simulink model "grid_following_dqctrl"  (R2026b)
settings: Solver=VariableStepAuto
undefined symbols (not defined in the file or in its folder): param
libraries: nesl_utility x2, afe_ssc_lib x1
settings Model: Creator=d.bagnara  LastModifiedBy=d.bagnara

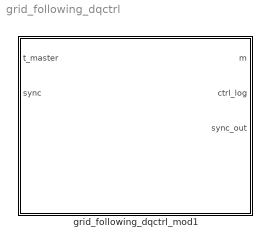
== system grid_following_dqctrl ==
  grid_following_dqctrl_mod1 : Subsystem  mask(Grid-following AFE (two-level bridge, LCL filter)){p=param.afe_follower(1)}
      mask prompts: p "Parameter struct p (afe_follower_module_param)"
      mask help: Grid-following AFE (DC-link voltage control, FHT-PLL) in one block: ideal two-level bridge, DC-link capacitor and LCL filter as a Simscape language component (afe_ssc.afe_two_level_lcl of afe_dq_single_block), control and PWM as one MATLAB Function (afe_follower_ctrl_pwm), measurements to the control through a Unit Delay of one tc (no algebraic loop). Interface of afe_dq_mod1 of grid_follower_dq.slx: ug_a/b/c left, Udc(+)/Udc(-) right, t_master in, M (14x1 pu) and ctrl_log (45x1) out. Master/slave: sync in and sync_out out, [i_xi_ref; i_eta_ref] in pu of ibez; with p.ctrl.slave = 1 the block runs its PLL and its current loops with the current references of the master (sync_out of the master to sync of the slave) and its DC-link loop is at rest, with p.ctrl.slave = 0 or absent it is a master and ignores sync. Parameter p: struct of private/afe_follower_module_param.m, e.g. param.afe_follower(1).
      mask Help: eval('pwrdoc = which(''grid_forming_following_afe.pdf''); if isempty(pwrdoc), pwrdoc = ''https://github.com/pwr-control/library/blob/main/library/documentation/grid_forming_following_afe/grid_forming_following_afe.pdf''; end; web(pwrdoc, ''-browser''); clear pwrdoc')
      mask Display:
      | port_label('LConn', 1, 'ug_a');
      | port_label('LConn', 2, 'ug_b');
      | port_label('LConn', 3, 'ug_c');
      | port_label('RConn', 1, 'Udc(+)');
      | port_label('RConn', 2, 'Udc(-)');
      | port_label('input', 1, 't_master');
      | port_label('input', 2, 'sync');
      | port_label('output', 1, 'M');
      | port_label('output', 2, 'ctrl_log');
      | port_label('output', 3, 'sync_out');

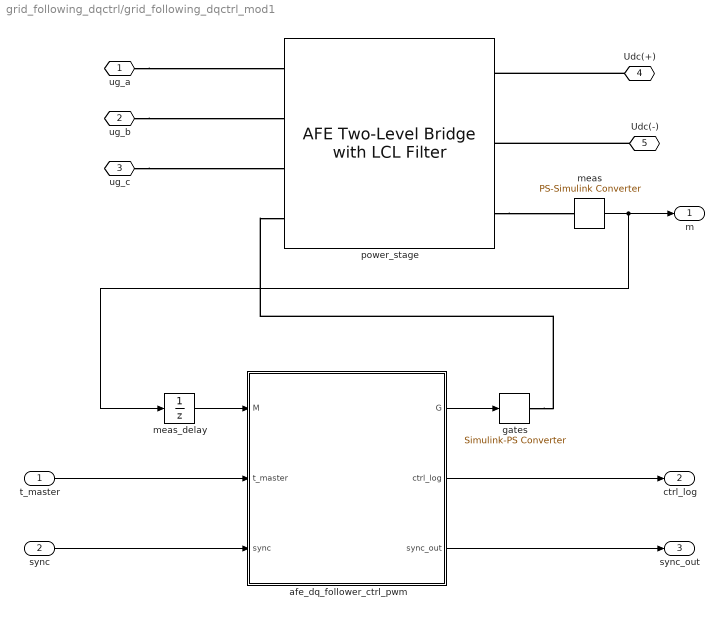
== system grid_following_dqctrl/grid_following_dqctrl_mod1 ==
  t_master : Inport
  sync : Inport  Port=2
  afe_dq_follower_ctrl_pwm : MATLAB Function  TreatAsAtomicUnit=on
  gates : nesl_utility/Simulink-PS Converter  PhysicalDomain=network_engine_domain  SubClassName=ps_input  LeftPortType=input  RightPortType=output  PseudoPeriodic=off  Frequencies=[]  NoiseDistribution=none  NoiseParameters=[]  Unit=V  AffineConversion=off  FilteringAndDerivatives=provide  SimscapeFilterOrder=1  InputFilterTimeConstant=0.001  UdotUserProvided=0
  meas : nesl_utility/PS-Simulink Converter  PhysicalDomain=network_engine_domain  SubClassName=ps_output  LeftPortType=input  RightPortType=output  PseudoPeriodic=off  Frequencies=[]  VectorFormat=inherit  Unit=1  AffineConversion=off
  meas_delay : UnitDelay  SampleTime=p.pwm.tc
  power_stage : afe_ssc_lib/AFE Two-Level Bridge with LCL Filter  Vth=p.hw.Vth V  Ron=p.hw.Ron Ohm  Goff=p.hw.Goff 1/Ohm  cap_dc=afe_ssc.onoff.on  Cdc=p.hw.Cdc F  Rdc=p.hw.Rdc Ohm  L1p=p.hw.L1p H  L10=p.hw.L10 H  R1=p.hw.R1 Ohm  Lls1=p.hw.Lls1 H  Cf=p.hw.Cf F  Rcf=p.hw.Rcf Ohm  L2p=p.hw.L2p H  L20=p.hw.L20 H  R2=p.hw.R2 Ohm  Lls2=p.hw.Lls2 H  ubez=p.hw.ubez V  ibez=p.hw.ibez A  udc_nom=p.hw.udc_nom V  vdc_specify=off  vdc_priority=None  vdc=0 V  vdc_nominal_specify=off  vdc_nominal_value=1  vdc_nominal_unit=V  vcap_specify=off  vcap_priority=None  vcap=0 V  vcap_nominal_specify=off  vcap_nominal_value=1  vcap_nominal_unit=V  ic_specify=off  ic_priority=None  ic=0 A  ic_nominal_specify=off  ic_nominal_value=1  ic_nominal_unit=A  vm_a_specify=off  vm_a_priority=None  vm_a=0 V  vm_a_nominal_specify=off  vm_a_nominal_value=1  vm_a_nominal_unit=V  vm_b_specify=off  vm_b_priority=None  vm_b=0 V  vm_b_nominal_specify=off  vm_b_nominal_value=1  vm_b_nominal_unit=V  vm_c_specify=off  vm_c_priority=None  vm_c=0 V  vm_c_nominal_specify=off  vm_c_nominal_value=1  vm_c_nominal_unit=V  i_ah_specify=off  i_ah_priority=None  i_ah=0 A  i_ah_nominal_specify=off  i_ah_nominal_value=1  i_ah_nominal_unit=A  i_al_specify=off  i_al_priority=None  i_al=0 A  i_al_nominal_specify=off  i_al_nominal_value=1  i_al_nominal_unit=A  i_bh_specify=off  i_bh_priority=None  i_bh=0 A  i_bh_nominal_specify=off  i_bh_nominal_value=1  i_bh_nominal_unit=A  i_bl_specify=off  i_bl_priority=None  i_bl=0 A  i_bl_nominal_specify=off  i_bl_nominal_value=1  i_bl_nominal_unit=A  i_ch_specify=off  i_ch_priority=None  i_ch=0 A  i_ch_nominal_specify=off  i_ch_nominal_value=1  i_ch_nominal_unit=A  i_cl_specify=off  i_cl_priority=None  i_cl=0 A  i_cl_nominal_specify=off  i_cl_nominal_value=1  i_cl_nominal_unit=A  i1_a_specify=off  i1_a_priority=None  i1_a=0 A  i1_a_nominal_specify=off  i1_a_nominal_value=1  i1_a_nominal_unit=A  i1_b_specify=off  i1_b_priority=None  i1_b=0 A  i1_b_nominal_specify=off  i1_b_nominal_value=1  i1_b_nominal_unit=A  i1_c_specify=off  i1_c_priority=None  i1_c=0 A  i1_c_nominal_specify=off  i1_c_nominal_value=1  i1_c_nominal_unit=A  vk_a_specify=off  vk_a_priority=None  vk_a=0 V  vk_a_nominal_specify=off  vk_a_nominal_value=1  vk_a_nominal_unit=V  vk_b_specify=off  vk_b_priority=None  vk_b=0 V  vk_b_nominal_specify=off  vk_b_nominal_value=1  vk_b_nominal_unit=V  vk_c_specify=off  vk_c_priority=None  vk_c=0 V  vk_c_nominal_specify=off  vk_c_nominal_value=1  vk_c_nominal_unit=V  vn_specify=off  vn_priority=None  vn=0 V  vn_nominal_specify=off  vn_nominal_value=1  vn_nominal_unit=V  vc_a_specify=off  vc_a_priority=None  vc_a=0 V  vc_a_nominal_specify=off  vc_a_nominal_value=1  vc_a_nominal_unit=V  vc_b_specify=off  vc_b_priority=None  vc_b=0 V  vc_b_nominal_specify=off  vc_b_nominal_value=1  vc_b_nominal_unit=V  vc_c_specify=off  vc_c_priority=None  vc_c=0 V  vc_c_nominal_specify=off  vc_c_nominal_value=1  vc_c_nominal_unit=V  i2_a_specify=off  i2_a_priority=None  i2_a=0 A  i2_a_nominal_specify=off  i2_a_nominal_value=1  i2_a_nominal_unit=A  i2_b_specify=off  i2_b_priority=None  i2_b=0 A  i2_b_nominal_specify=off  i2_b_nominal_value=1  i2_b_nominal_unit=A  i2_c_specify=off  i2_c_priority=None  i2_c=0 A  i2_c_nominal_specify=off  i2_c_nominal_value=1  i2_c_nominal_unit=A  j_ab_specify=off  j_ab_priority=None  j_ab=0 A  j_ab_nominal_specify=off  j_ab_nominal_value=1  j_ab_nominal_unit=A  j_bc_specify=off  j_bc_priority=None  j_bc=0 A  j_bc_nominal_specify=off  j_bc_nominal_value=1  j_bc_nominal_unit=A
  ug_a : PMIOPort  Side=Left
  ug_b : PMIOPort  Port=2  Side=Left
  ug_c : PMIOPort  Port=3  Side=Left
  Udc(+) : PMIOPort  Port=4  Side=Right
  Udc(-) : PMIOPort  Port=5  Side=Right
  m : Outport
  ctrl_log : Outport  Port=2
  sync_out : Outport  Port=3
  wires:
  t_master/1 -> afe_dq_follower_ctrl_pwm/2(t_master)
  meas/1 -> m/1, meas_delay/1
  meas_delay/1 -> afe_dq_follower_ctrl_pwm/1(M)
  afe_dq_follower_ctrl_pwm/1(G) -> gates/1
  afe_dq_follower_ctrl_pwm/2(ctrl_log) -> ctrl_log/1
  sync/1 -> afe_dq_follower_ctrl_pwm/3(sync)
  afe_dq_follower_ctrl_pwm/3(sync_out) -> sync_out/1
  connections:
  gates/RConn1 -- power_stage/LConn4
  power_stage/RConn3 -- meas/LConn1
  ug_a/RConn1 -- power_stage/LConn1
  ug_b/RConn1 -- power_stage/LConn2
  ug_c/RConn1 -- power_stage/LConn3
  Udc(+)/RConn1 -- power_stage/RConn1
  Udc(-)/RConn1 -- power_stage/RConn2

== matlab function grid_following_dqctrl/grid_following_dqctrl_mod1/afe_dq_follower_ctrl_pwm ==
  settings: updateMethod=DISCRETE  sampleTime=p.pwm.tc
  data: M input; G output; t_master input; sync input size=[2 1]; ctrl_log output; p parameter; sync_out output size=[2 1]
function [G, ctrl_log, sync_out] = afe_follower_ctrl_pwm(M, t_master, sync, p)
%AFE_FOLLOWER_CTRL_PWM  Control and PWM of one grid-following AFE (DC-link voltage control) in one MATLAB Function block.
%#codegen
%
%   [G, ctrl_log, sync_out] = afe_follower_ctrl_pwm(M, t_master, sync, p)
%
%   Equivalent of afe_dq_mod1/AFE_control (triggered subsystem afe_control) plus afe/sv_pwm (carrier,
%   TRGO, gate commands) of grid_follower_dq.slx (R2026b, commit 3fa4567), written as one function so
%   that the control of one AFE counts as ONE nonvirtual block (MATLAB Home licence: 1000 nonvirtual
%   blocks per model, referenced models and library links included). Same structure as
%   afe_dq_ctrl_pwm.m of ../afe_dq_single_block (grid-forming AFE): the block runs at the fixed sample
%   time p.pwm.tc, the step of the Simscape local solver; the control runs on the rising edge of the
%   TRGO flag derived from the carrier of the local clock, exactly as the triggered subsystem.
%
%   Inputs
%     M        measurement vector [14x1] in pu of the block afe_ssc.afe_two_level_lcl:
%              M(1:3) is_abc converter current (positive out of the bridge), M(4:6) uc_abc filter
%              capacitor voltage, M(7:9) ig_abc grid current (positive towards the grid),
%              M(10:12) ug_abc grid voltage without zero sequence, M(13) vdc/udc_nom, M(14) ic/ibez
%     t_master master time [s] (Clock of "global timing"/time_afe3 with k = 1, i.e. simulation time)
%     sync     [2x1] [i_xi_ref; i_eta_ref] of the master (its output sync_out), read only in slave mode
%              (p.ctrl.slave = 1); on a master leave it unconnected or grounded
%     p        parameter struct, scope "Parameter" in the Symbols pane of the block, built by
%              private/afe_follower_module_param.m (p.pwm.*, p.ctrl.*); p.ctrl.slave (optional, default 0)
%              selects the slave mode
%   Outputs
%     G        gate commands [6x1] in V, order [a+; a-; b+; b-; c+; c-] (Q1..Q6 of the PWM library
%              block and G of the ssc block), p.pwm.gate_on / p.pwm.gate_off (15 V / -10 V)
%     ctrl_log control signals [45x1], indices in afe_follower_log_index.m (held between two
%              triggers; t_loc, ramp and trgo updated every step)
%     sync_out [2x1] [i_xi_ref; i_eta_ref] of the last control step (held between two triggers), in pu
%              of ibez: connect it to the input sync of the slave(s)
%
%   Master/slave (p.ctrl.slave = 1): converters in parallel on one DC link. The master (p.ctrl.slave
%   absent or 0) runs the DC-link voltage loop; a slave takes the current references of the master from
%   sync, saturated at +-ixi_lim, and runs its own PLL, current loops and modulator, so that the modules
%   carry the same current in pu of their own ibez. The DC-link PI of a slave is at rest (its reference
%   filter and its error are still computed for the log). With one DC-link loop per module on the same
%   capacitors only the sum of the module currents is defined: any difference between the DC-link
%   acquisitions of two modules is integrated into a difference of current. Master and slaves with the
%   same clock and carrier phase run in the same tc step, the master first (data dependency), so a slave
%   uses the references of the same trigger; with a carrier phase shift it uses those of the last one.
%
%   Chain reproduced (names of the blocks of grid_follower_dq.slx in brackets):
%     every step tc
%       local clock    t_loc = t_master*k_time*(1 + corr)              [global timing/time_afe1]
%       carrier        ramp = asin(sin(2*pi*fpwm*t_loc - phase - pi/2))/pi + 1/2   [ramp_up_down]
%       TRGO           ramp <= 2*fpwm*tc or ramp >= 1 - 2*fpwm*tc (double update)  [trgo_gen]
%       gates          upper on: ramp >= d + dead_time*fpwm, lower on: ramp <= d - dead_time*fpwm,
%                      d saturated in [m_low, m_up]                    [gate commands]
%     on the rising edge of TRGO (no trigger on the first evaluation, as the Trigger block)
%       acquisitions   quantizer (adc_q) and one-step delay of ug, is, ig (ig with gain -1), udc
%                      [acquisitions/* quantizzation and one step delay]; the grid-emulator phase
%                      acquisition (grid_phase_acquisition) is a log only and is not reproduced
%       alignment      PI of (t_master - t_loc), saturated, back-calculation anti-windup, output
%                      corr applied from the next step                [phase_compensation_1]
%       FHT            first harmonic tracker on ug_alpha and ug_beta (port of
%                      first_harmonic_tracker.c, reset while t_master < fht_t_reset), "positive
%                      sequence" with the gains seq_gain (-1/2 in the model) [filter_and_transformation]
%       PLL stage A    |u| = sqrt(ualpha^2 + ubeta^2) saturated at u_mag_min, 1/|u| (Vgrid_unorm_fht),
%                      alpha/beta -> xi/eta with the PLL angle of the previous step  [pll_stageA]
%       PLL stage B    e = pll_err_sign*u_eta/|u| (Product1, Gain -1), PI (pll_p, pll_i1*ts) in pu of
%                      omega_nom, gamma += ts*omega_nom*(P + I), wrapped to [-pi, pi) (bounder1);
%                      double integrator observer on gamma for the omega estimate (log only)
%                      [pll_stageB, double_integrator_observer]
%       udc loop       udc_ref = low-pass (tau = udc_tau) of the Step udc_norm_ref at udc_t_step
%                      [discrete-time-low-pass-filter1, udc_norm_ref], PI (kp_udc, ki_udc*ts) on
%                      udc_ref - udc with saturation +-ixi_lim and back-calculation, i_xi_ref = -y
%                      [udc_ctrl]; i_eta_ref = ieta_ref (Constant 0 of current_ctrl); a slave takes
%                      i_xi_ref and i_eta_ref of the master from sync
%       current loop   dq vector PI on (i_xi, i_eta), unit-circle limiter   [current_ctrl]
%       zero sequence  iz = (is_a + is_b + is_c)/3, PI (kp_iz, ki_iz*ts), saturation +-iz_lim,
%                      back-calculation, gain iz_out_gain -> ugamma   [zero_current_ctrl]
%       SVPWM          port of sv_pwm_cm.c (inputs scaled by sqrt(3)/2, k_offset = (ugamma*u_cm + 1)/2)
%                      [space_vector]
%
%   Signs (see README.md, section 4.2): the model has the positive-sequence gains -1/2 (the sign
%   corrected in grid_forming_dq by commit e61afe1) AND the PLL error -u_eta/|u|; the two errors
%   cancel and the PLL locks on the true grid angle. p.ctrl.seq_gain and p.ctrl.pll_err_sign carry
%   both signs so that the code follows the model as it is (-1/2, -1) or the corrected pair (+1/2, +1);
%   changing only one of them makes the PLL lock 180 degrees off and the DC-link loop diverge.
%
%   Differences from the block diagram (same as the grid-forming version, README.md section 6):
%     - the duties change at the trigger step without the 1/(tc*s + 1) filters td2tc_1..3
%     - the switching instants are quantized to tc; the ramp of the trigger step is used for the gates
%     - double precision instead of the single precision of the C-Caller blocks

NLOG = 45;

persistent initialized trgo_z corr_z x_align ug_z is_z ig_z udc_z ...
           fht_s1 fht_s2 fht_out gam pll_i1 x_obs udc_step_z udc_ref_z x_udc ...
           xd_i xq_i clip_i_z x_iz d_abc logv sync_z

if isempty(initialized)
    initialized = true;
    trgo_z   = true;                 % Trigger block "compatibility (no trigger on first evaluation)"
    corr_z   = 0;                    % local time correction (Unit Delay of "global timing")
    x_align  = 0;                    % integrator of the alignment PI
    ug_z     = zeros(3,1);           % one-step delays of the acquisitions
    is_z     = zeros(3,1);
    ig_z     = zeros(3,1);
    udc_z    = 0;
    fht_s1   = zeros(2,1);           % FHT state 1, [alpha; beta]
    fht_s2   = zeros(2,1);           % FHT state 2
    fht_out  = zeros(2,1);           % FHT output (state 1 of the previous step)
    gam      = 0;                    % PLL angle (Unit Delay1/Unit Delay2 of pll_stageB)
    pll_i1   = 0;                    % integrator of the PLL PI (Unit Delay4 of pll_stageB), pu of omega_nom
    x_obs    = zeros(2,1);           % double integrator observer state [theta_hat; omega_hat] (Unit Delay)
    udc_step_z = 0;                  % Unit Delay of the low-pass filter input (Step udc_norm_ref)
    udc_ref_z  = 0;                  % Unit Delay1 of the low-pass filter output
    x_udc    = 0;                    % integrator of the DC-link PI (Unit Delay4 of udc_ctrl)
    xd_i = 0; xq_i = 0; clip_i_z = 0;      % current loop PI
    x_iz     = 0;                    % integrator of the zero-sequence PI (Unit Delay4)
    d_abc    = zeros(3,1);           % duties before the first trigger (Outport initial output)
    logv     = zeros(NLOG,1);
    sync_z   = zeros(2,1);           % [i_xi_ref; i_eta_ref] of the last trigger (output sync_out)
end

m = M(:);
slave = false;                       % p.ctrl.slave is optional: parameter structs of older models have none
if isfield(p.ctrl, 'slave')
    slave = p.ctrl.slave ~= 0;
end

% ------------------------------------------------------------------ every step: local clock, carrier, TRGO
t_loc = t_master*p.ctrl.k_time*(1 + corr_z);
ramp  = asin(sin(2*pi*p.pwm.fpwm*t_loc - p.pwm.phase - pi/2))/pi + 1/2;
th_trgo = p.pwm.fpwm*p.pwm.tc*2;
if p.pwm.double_update ~= 0
    trgo = (ramp >= 0 && ramp <= th_trgo) || (ramp <= 1 && ramp >= 1 - th_trgo);
else
    trgo = (ramp >= 0 && ramp <= th_trgo);
end

if trgo && ~trgo_z
    % ============================================================== control step (triggered subsystem)
    ts   = p.ctrl.ts;                % control sample time (ts_afe)
    ts_i = p.ctrl.ts_int;            % sample time of the current-loop PI integrators (ts_inv in the model, = ts_afe)

    % ---- acquisitions: the control uses the samples of the previous trigger (Unit Delay after the
    %      Quantizer), the delay states take the samples of this trigger
    ugd  = ug_z;
    isd  = is_z;
    igd  = ig_z;
    udcd = udc_z;
    q = p.ctrl.adc_q;
    ug_z  = q*round(m(10:12)/q);
    is_z  = q*round(m(1:3)/q);
    ig_z  = -q*round(m(7:9)/q);      % Gain -1 after the delay ("ig afe quantizzation and one step delay")
    udc_z = q*round(m(13)/q);

    % ---- alignment of the local clock to the master time (phase_compensation_1/alignment_eval_afe1/pi)
    e_al = t_master - t_loc;         % u_ref - u with u_ref = 0, u = -(master - local)
    P_al = p.ctrl.kp_align*e_al;
    y_al = P_al + p.ctrl.ki_align*ts*e_al + x_align;
    y_al = min(max(y_al, p.ctrl.lim_down_align), p.ctrl.lim_up_align);
    x_align = y_al - P_al;           % Sum3 -> Unit Delay4 (back-calculation anti-windup)
    corr_z  = y_al;                  % Goto local_time_corr_afe1, applied from the next step

    % ---- grid voltage: abc -> alpha/beta (abc2alphabeta), FHT, "positive sequence"
    ug_alpha = 2/3*(ugd(1) - 1/2*ugd(2) - 1/2*ugd(3));
    ug_beta  = 1/sqrt(3)*(ugd(2) - ugd(3));
    reset = t_master < p.ctrl.fht_t_reset;             % Step block of FHTalpha/FHTbeta: 1 until fht_t_reset
    w  = p.ctrl.fht_omega;
    dl = p.ctrl.fht_delta;
    a_ = -w*w;
    b_ = -dl*w;
    a11 = 1 + 0.5*a_*ts*ts;                            % first_harmonic_tracker_init
    a12 = ts + 0.5*b_*ts*ts;
    a21 = a_*ts + 0.5*a_*b_*ts*ts;
    a22 = 1 + b_*ts + 0.5*(a_ + b_*b_)*ts*ts;
    l1 = p.ctrl.fht_l1;
    l2 = p.ctrl.fht_l2;
    u_in  = [ug_alpha; ug_beta];
    u_hat = zeros(2,1);
    v_hat = zeros(2,1);
    for ch = 1:2
        if reset                                       % reset reloads the instance: states and output to zero
            fht_s1(ch)  = 0;
            fht_s2(ch)  = 0;
            fht_out(ch) = 0;
        end
        err = u_in(ch) - fht_out(ch);                  % first_harmonic_tracker_process
        s1n = l1*err + a11*fht_s1(ch) + a12*fht_s2(ch);
        s2n = l2*err + a21*fht_s1(ch) + a22*fht_s2(ch);
        fht_out(ch) = fht_s1(ch);                      % output = c1*state1 before the update
        fht_s1(ch)  = s1n;
        fht_s2(ch)  = s2n;
        u_hat(ch) = fht_out(ch);                       % output_pu_hat
        v_hat(ch) = fht_s2(ch)/w;                      % output_pu_hat_dot * (1/omega_fht)
    end
    u_fhtsr_alpha = p.ctrl.seq_gain*(u_hat(1) + v_hat(2));   % Sum (++): u_fht_alpha + v_fht_beta, Gain seq_gain (-1/2 in the model)
    u_fhtsr_beta  = p.ctrl.seq_gain*(u_hat(2) - v_hat(1));   % Sum1 (-+): -v_fht_alpha + u_fht_beta, Gain1 seq_gain
    u_grid_mag = sqrt(u_fhtsr_alpha^2 + u_fhtsr_beta^2);     % Math Function (magnitude^2) x2, Sum, Sqrt
    u_inv = 1/max(u_grid_mag, p.ctrl.u_mag_min);             % Saturation (lower limit 0.02), Reciprocal Sqrt -> Vgrid_unorm_fht

    % ---- PLL stage A: rotating frame with the PLL angle of the previous step (sequences/alphabeta2xieta_pos)
    gamma = gam;                                       % Unit Delay2 of pll_stageB (same value as Unit Delay1)
    u_xi  =  u_fhtsr_alpha*cos(gamma) + u_fhtsr_beta*sin(gamma);
    u_eta = -u_fhtsr_alpha*sin(gamma) + u_fhtsr_beta*cos(gamma);

    % ---- PLL stage B: PI on the normalized eta component, angle integration, wrap (pll_stageB)
    e_pll  = p.ctrl.pll_err_sign*u_eta*u_inv;         % Product1 (u_eta * 1/|u|), Gain -1 in the model
    pll_i1 = pll_i1 + p.ctrl.pll_i1*ts*e_pll;         % Sum3 "i1": kp (pll_i1_fht*ts) + Unit Delay4
    omega_pu = p.ctrl.pll_p*e_pll + pll_i1;           % Sum5: kp1 (pll_p_fht) + i1, pu of omega_nom
    gam = wrap_pi(gamma + ts*p.ctrl.omega_nom*omega_pu);   % Product2 (omega_nom), kp2 (ts), Sum4, bounder1

    % ---- double integrator observer on the PLL angle: omega estimate for the log (double_integrator_observer)
    theta_hat = wrap_pi(p.ctrl.obs_C*x_obs);          % Gain2 (Cso), bounder2
    e_obs = wrap_pi(gamma - theta_hat);                % Sum "e" (-+), bounder1
    omega_hat = x_obs(2);                              % Selector (index 2) of the Unit Delay output
    x_obs = p.ctrl.obs_A*x_obs + p.ctrl.obs_L*e_obs;   % Gain1 (Adso) + Gain (Ldso) -> Unit Delay
    omega_pll_pu = omega_hat/p.ctrl.omega_nom;         % kp3 (1/omega_grid_nom)

    % ---- DC-link voltage loop (udc_ctrl): reference step through the discrete low-pass filter, PI
    step_now = double(t_master >= p.ctrl.udc_t_step)*p.ctrl.udc_norm_ref;    % Step udc_norm_ref (Time 1e-3)
    a_lpf = ts/p.ctrl.udc_tau;                                               % discrete-time-low-pass-filter1 (tau 20e-3)
    udc_ref = a_lpf*udc_step_z + (1 - a_lpf)*udc_ref_z;                      % y(k) = ts/tau*x(k-1) + (1 - ts/tau)*y(k-1)
    udc_step_z = step_now;
    udc_ref_z  = udc_ref;
    e_udc = udc_ref - udcd;                            % Sum2 (-+): udc_pu_ref - udc_pu (acquired, one-step delayed)
    P_udc = p.ctrl.kp_udc*e_udc;                       % Gain "1/Ti" = kp_udc_ctrl
    if slave
        % slave: current references of the master, DC-link PI at rest
        i_xi_ref  = min(max(sync(1), -p.ctrl.ixi_lim), p.ctrl.ixi_lim);
        i_eta_ref = sync(2);
        sat_udc = double(i_xi_ref ~= sync(1));
        x_udc = 0;
    else
        y_udc = P_udc + p.ctrl.ki_udc*ts*e_udc + x_udc;    % Sum1 (+++): P, "kp" = ki_udc_ctrl*ts_afe, Unit Delay4
        y_sat = min(max(y_udc, -p.ctrl.ixi_lim), p.ctrl.ixi_lim);           % Saturation +-ixi_pos_ref_lim
        x_udc = y_sat - P_udc;                             % Sum3 (-+) -> Unit Delay4 (back-calculation anti-windup)
        sat_udc = double(y_sat ~= y_udc);
        i_xi_ref  = -y_sat;                                % Gain -1: current OUT of the bridge negative when the DC link must charge
        i_eta_ref = p.ctrl.ieta_ref;                       % Constant of current_ctrl (0)
    end

    % ---- current loop (current_ctrl): converter current in the PLL frame, dq vector PI
    i_alpha = 2/3*(isd(1) - 1/2*isd(2) - 1/2*isd(3));  % uvw2alphabeta
    i_beta  = 2/3*(sqrt(3)/2*(isd(2) - isd(3)));
    i_xi  =  i_alpha*cos(gamma) + i_beta*sin(gamma);   % alphabeta2xieta with phase_grid_pll
    i_eta = -i_alpha*sin(gamma) + i_beta*cos(gamma);
    [m_d, m_q, clip_i, xd_i, xq_i] = dq_vector_pi( ...
        i_xi_ref - i_xi, i_eta_ref - i_eta, xd_i, xq_i, clip_i_z, ...
        p.ctrl.kp_i, p.ctrl.ki_i*ts_i, p.ctrl.clip_release*ts_i, p.ctrl.u_lim, p.ctrl.u_lim);
    clip_i_z = clip_i;
    u_alpha = m_d*cos(gamma) - m_q*sin(gamma);         % xi_eta_to_alpha_beta
    u_beta  = m_d*sin(gamma) + m_q*cos(gamma);

    % ---- zero-sequence current loop (zero_current_ctrl/iz, zero_sequence_current_ctrl)
    iz = (isd(1) + isd(2) + isd(3))/3;                 % Sum (+++), Gain 1/3
    e_iz = p.ctrl.iz_ref - iz;                         % Sum2 (-+): iz_pu_ref - iz_pu
    P_iz = p.ctrl.kp_iz*e_iz;                          % Gain "1/Ti" = kp_is_z
    y_iz = P_iz + p.ctrl.ki_iz*ts*e_iz + x_iz;         % Sum1 (+++): P, "kp" = ki_is_z*ts_afe, Unit Delay4
    y_iz = min(max(y_iz, -p.ctrl.iz_lim), p.ctrl.iz_lim);   % Saturation +-1
    x_iz = y_iz - P_iz;                                % Sum3 (-+) -> Unit Delay4
    u_gamma = p.ctrl.iz_out_gain*y_iz;                 % Gain (1) -> ugamma_ctrl_afe

    % ---- space vector modulator (space_vector: gains sqrt(3)/2, u_cm_comp, C Caller sv_pwm_cm)
    [da, db, dc] = sv_pwm_cm(u_alpha*sqrt(3)/2, u_beta*sqrt(3)/2, u_gamma*p.ctrl.u_cm, true);
    d_abc = [da; db; dc];

    % ---- log (indices: afe_follower_log_index.m)
    logv(4)  = corr_z;
    logv(5)  = gamma;
    logv(6)  = omega_pll_pu;
    logv(7:9)   = ugd;
    logv(10:12) = isd;
    logv(13:15) = igd;
    logv(16) = udcd;
    logv(17) = u_fhtsr_alpha;
    logv(18) = u_fhtsr_beta;
    logv(19) = u_grid_mag;
    logv(20) = u_xi;
    logv(21) = u_eta;
    logv(22) = e_pll;
    logv(23) = pll_i1;
    logv(24) = udc_ref;
    logv(25) = e_udc;
    logv(26) = i_xi_ref;
    logv(27) = i_eta_ref;
    logv(28) = sat_udc;
    logv(29) = i_xi;
    logv(30) = i_eta;
    logv(31) = m_d;
    logv(32) = m_q;
    logv(33) = clip_i;
    logv(34) = u_alpha;
    logv(35) = u_beta;
    logv(36) = iz;
    logv(37) = u_gamma;
    logv(38:40) = d_abc;
    logv(41) = u_hat(1);
    logv(42) = v_hat(1);
    logv(43) = u_hat(2);
    logv(44) = v_hat(2);
    logv(45) = theta_hat;

    % ---- references for the slave(s)
    sync_z = [i_xi_ref; i_eta_ref];
end
trgo_z = trgo;

% ------------------------------------------------------------------ every step: gate commands
dtf = p.pwm.dead_time*p.pwm.fpwm;                      % dead time as a fraction of the carrier period
G = p.pwm.gate_off*ones(6,1);
for k = 1:3
    dk = min(max(d_abc(k), p.pwm.m_low), p.pwm.m_up);  % Saturation m_low..m_up
    if ramp >= dk + dtf                                % upper switch: (m + dead_time*f) <= ramp
        G(2*k-1) = p.pwm.gate_on;
    end
    if ramp <= dk - dtf                                % lower switch: ramp <= (m - dead_time*f)
        G(2*k) = p.pwm.gate_on;
    end
end

logv(1) = t_loc;
logv(2) = ramp;
logv(3) = double(trgo);
ctrl_log = logv;
sync_out = sync_z;

end

% ======================================================================================================
function y = wrap_pi(u)
%WRAP_PI  Port of the MATLAB Function "bounder" of the model: y = -pi + mod(u + 3*pi, 2*pi), i.e. [-pi, pi).
    y = -pi + mod(u + 3*pi, 2*pi);
end

% ======================================================================================================
function [md_sat, mq_sat, clip, xd, xq] = dq_vector_pi(ed, eq, xd, xq, clip_z, kp, ki_ts, rel_ts, lim, clip_thr)
%DQ_VECTOR_PI  dq vector PI of the model: blocks pi_d, pi_q, "vector lenght", bounder1/2, switch.
%   ed, eq      errors (reference - measure)
%   xd, xq      integrator states (Unit Delay2 of pi_d, pi_q)
%   clip_z      clip flag of the previous step (Unit Delay1 of pi_d, pi_q)
%   kp, ki_ts   proportional gain and integral gain already multiplied by the sample time
%   rel_ts      CTRPIFF_CLIP_RELEASE*ts, leak of the integrator while clipped
%   lim         radius of the output limiter (Switch1 threshold and gain of the bounders)
%   clip_thr    radius at which the clip flag is raised (Switch threshold of the bounders)
    if clip_z > 0.5
        xd_new = xd - rel_ts*xd;                       % Sum2: x - rel*ts*x
        md = kp*ed + xd;                               % Sum5 = P + Sum4, Sum4 = x + 0
        xq_new = xq - rel_ts*xq;
        mq = kp*eq + xq;
    else
        xd_new = xd + ki_ts*ed;                        % Sum4 = x + ki*ts*e
        md = kp*ed + xd_new;
        xq_new = xq + ki_ts*eq;
        mq = kp*eq + xq_new;
    end
    xd = xd_new;
    xq = xq_new;
    mag = sqrt(md^2 + mq^2);                           % "vector lenght"
    if mag >= lim                                      % bounder1/2: Switch1 (u2 >= Threshold)
        md_sat = md/mag*lim;
        mq_sat = mq/mag*lim;
    else
        md_sat = md;
        mq_sat = mq;
    end
    if mag >= clip_thr                                 % bounder1/2: Switch (u2 >= Threshold), OR in "switch"
        clip = 1;
    else
        clip = 0;
    end
end

% ======================================================================================================
function [da, db, dc] = sv_pwm_cm(ualpha, ubeta, ugamma, enable)
%SV_PWM_CM  Port of sv_pwm_cm_process (library/user_defined_functions/ccaller/src/sv_pwm_cm.c).
%   Duties da, db, dc in [0, 1] are the switch-on instants on the carrier (0 = bottom, 1 = top):
%   the upper switch is on while ramp >= d. k_offset = 0.5 is the standard SVPWM, 0 only V0,
%   1 only V7. The overmodulation branch of the C code (t0 < 0) computes the same expressions
%   as the linear branch, so it is not repeated here.
    k_offset = (ugamma + 1)/2;
    sq3 = sqrt(3);
    if enable
        angle = atan2(ubeta, ualpha);
        if angle >= 0 && angle <= pi/3                 % sector 1
            t2 = ubeta*2/sq3;
            t1 = ualpha - ubeta/sq3;
            t0 = 1 - t2 - t1;
            da = t0*k_offset;
            db = t1 + da;
            dc = t2 + db;
        elseif angle >= pi/3 && angle <= 2*pi/3        % sector 2
            t1 = -ualpha + ubeta/sq3;
            t2 = ualpha + ubeta/sq3;
            t0 = 1 - t2 - t1;
            db = t0*k_offset;
            da = t1 + db;
            dc = t2 + da;
        elseif angle >= 2*pi/3 && angle <= pi          % sector 3
            t2 = -ubeta/sq3 - ualpha;
            t1 = ubeta*2/sq3;
            t0 = 1 - t2 - t1;
            db = t0*k_offset;
            dc = t1 + db;
            da = t2 + dc;
        elseif angle >= -pi && angle <= -2*pi/3        % sector 4
            t1 = -2/sq3*ubeta;
            t2 = ubeta/sq3 - ualpha;
            t0 = 1 - t2 - t1;
            dc = t0*k_offset;
            db = t1 + dc;
            da = t2 + db;
        elseif angle >= -2*pi/3 && angle <= -pi/3      % sector 5
            t2 = ualpha - ubeta/sq3;
            t1 = -ualpha - ubeta/sq3;
            t0 = 1 - t2 - t1;
            dc = t0*k_offset;
            da = t1 + dc;
            db = t2 + da;
        else                                           % sector 6
            t1 = ualpha + ubeta/sq3;
            t2 = -ubeta*2/sq3;
            t0 = 1 - t2 - t1;
            da = t0*k_offset;
            dc = t1 + da;
            db = t2 + dc;
        end
    else
        da = 0.5;
        db = 0.5;
        dc = 0.5;
    end
end
